simulink model "PMSM_Simulation_2025a"  (R2025a)
settings: Solver=FixedStepDiscrete  StartTime=0.0  StopTime=10  FixedStep=0.00005/200  RelTol=1e-3
values from neighbouring files (symbols this model uses):
  MC_DCurrLopKi_CFG = 0.008293758    [PMSM_MC_Data_2025a.sldd]
  MC_DCurrLopKp_CFG = 0.0870848    [PMSM_MC_Data_2025a.sldd]
  MC_MotModeDebug_CFG = 255.0    [PMSM_MC_Data_2025a.sldd]
  MC_POLE_NUM_CFG = 7.0    [PMSM_MC_Data_2025a.sldd]
  MC_QCurrLopKi_CFG = 0.008293758    [PMSM_MC_Data_2025a.sldd]
  MC_QCurrLopKp_CFG = 0.0870848    [PMSM_MC_Data_2025a.sldd]
  MC_SpdLopKi_CFG = 1.0E-5    [PMSM_MC_Data_2025a.sldd]
  MC_SpdLopKp_CFG = 0.002    [PMSM_MC_Data_2025a.sldd]
undefined symbols (not defined in the file or in its folder): Ls, magnitude, Rs
libraries: simulink x28, slpidlib x6, spsDCVoltageSourceLib x1, spsPermanentMagnetSynchronousMachineLib x1, spsUniversalBridgeLib x1, sps_lib x1
(part 1 of 3)
settings Model: DataDictionary=PMSM_MC_Data_2025a.sldd  SimulationMode=accelerator  PacingRate=1000  Creator=EDY  LastModifiedBy=xiaoy
settings RTWCC: GPUComputeCapability=3.5

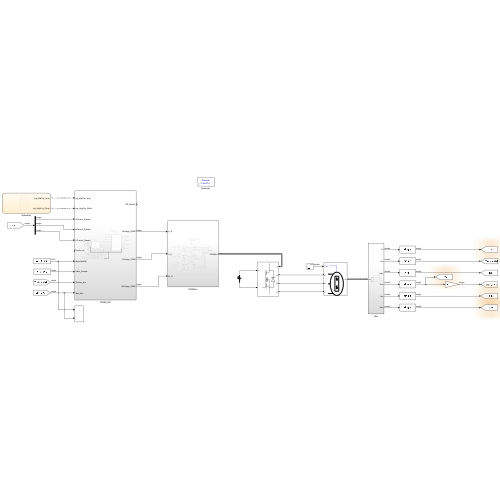
[thumbnail: Simulink's stored preview of the top-level diagram]
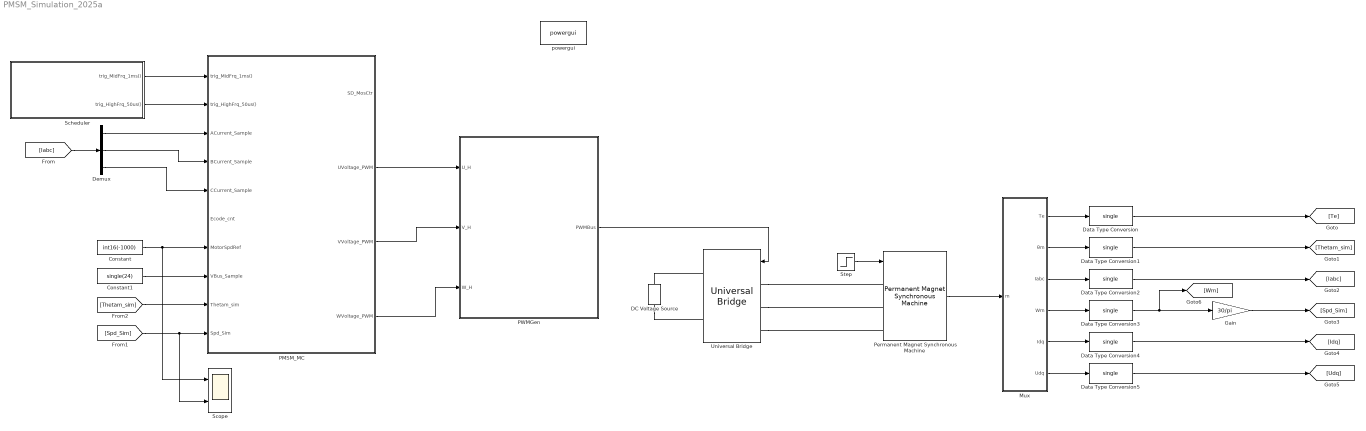
== system PMSM_Simulation_2025a ==
  Constant : Constant  Value=int16(-1000)
  Constant1 : Constant  Value=single(24)
  DC Voltage Source : spsDCVoltageSourceLib/DC Voltage Source  Amplitude=24  Measurements=None
  Data Type Conversion{,1..5} (6 alike) : DataTypeConversion  OutDataTypeStr=single  SaturateOnIntegerOverflow=off  RndMeth=Floor
  Demux : Demux  Outputs=3
  Gain : Gain  Gain=30/pi
  Mux : Subsystem
  PMSM_MC : Subsystem
  PWMGen : Subsystem
  Permanent Magnet Synchronous Machine : spsPermanentMagnetSynchronousMachineLib/Permanent Magnet Synchronous Machine  NbPhases=3  FluxDistribution=Sinusoidal  RotorType=Salient-pole  MechanicalLoad=Torque Tm  PresetModel=No  ShowDetailedParameters=on  MeasurementBus=off  Resistance=0.08  Inductance=8.5e-3  dqInductances=[0.000042,0.000042]  La=0.000395  MachineConstant=Flux linkage established by magnets (V.s)  Flux=0.00838  VoltageCst=10.6397  TorqueCst=0.08799  Flat=120  Mechanical=[0.000008 0 7 0]  PolePairs=4  InitialConditions=[0,0, 0,0]  InitialConditions5ph=[0 0 0 0 0 0]  RefAngle=Aligned with phase A axis (original Park)  IterativeDiscreteModel=Trapezoidal non iterative  TsBlock=-1  TsPowergui=0
  Scheduler : Stateflow chart  TreatAsAtomicUnit=on
  Scope : Scope  NumInputPorts=2
      settings: ActiveDisplayYMinimum=-1203.7366380691528  ActiveDisplayYMaximum=224.12290668487546
  Step : Step  Time=0  After=0  SampleTime=0
  Universal Bridge : spsUniversalBridgeLib/Universal Bridge  Arms=3  SnubberResistance=1e5  SnubberCapacitance=inf  Device=MOSFET / Diodes  Ron=1e-3  Lon=0  ForwardVoltages="[  0  0  ]"  ForwardVoltage=0  GTOparameters=[ 10e-6 , 20e-6 ]  IGBTparameters=[ 1e-6 , 2e-6 ]  Measurements=None  Measurements_2=None  converterType=Rectifier
  powergui : sps_lib/powergui  Priority=1  SimulationMode=Discrete  SampleTime=0.00005/200  frequency=60  Iterations=50  frequencyindice=0  Pbase=100e6  ErrMax=1e-4  UnitsV=kV  UnitsW=MW  buscounter=0  FunctionMessages=off  echomessages=off  EnableUseOfTLC=off  CurrentSourceSwitches=off  DisableSnubberDevices=off  DisableRonSwitches=off  DisableVfSwitches=off  DisplayEquations=off  AutomaticDiscreteSolvers=off  SolverType=Tustin/Backward Euler (TBE)  Interpol=off  ExternalGateDelay=off  methode=off  Ts=100  x0status=blocks  SPID=on  SwTol=0  HookPort=off  NonlinearTolerance=1e-4  nMaxIteration=100  ContinueOnMaxIteration=off  RestoreLinks=warning  ResistiveCurrentMeasurement=off  Frange=[0:2:500]  Ylog=off  Xlog=on  ShowGrid=off  save=off  variable=ZData  structure=0  ZoomFFT=off  StartTime=0.0  cycles=1  DisplayStyle=1  fundamental=60  FreqAxis=off  MaxFrequency=1000  frequencyindicesteady=1  RmsSteady=1  display=off
  wires:
  Step/1 -> Permanent Magnet Synchronous Machine/1
  Scheduler/1(trig_MidFrq_1ms()) -> PMSM_MC/1(trig_MidFrq_1ms())
  Scheduler/2(trig_HighFrq_50us()) -> PMSM_MC/2(trig_HighFrq_50us())
  PMSM_MC/2(UVoltage_PWM) -> PWMGen/1(U_H)
  PMSM_MC/3(VVoltage_PWM) -> PWMGen/2(V_H)
  PMSM_MC/4(WVoltage_PWM) -> PWMGen/3(W_H)
  PWMGen/1(PWMBus) -> Universal Bridge/1
  Permanent Magnet Synchronous Machine/1 -> Mux/1(m)
  Mux/1(Te) -> Data Type Conversion/1
  Mux/2(θm) -> Data Type Conversion1/1
  Mux/3(Iabc) -> Data Type Conversion2/1
  Mux/4(Wm) -> Data Type Conversion3/1
  Mux/5(Idq) -> Data Type Conversion4/1
  Mux/6(Udq) -> Data Type Conversion5/1
  Data Type Conversion/1 -> [Te]
  Data Type Conversion1/1 -> [Thetam_sim]
  Data Type Conversion2/1 -> [Iabc]
  Data Type Conversion3/1 -> Gain/1, [Wm]
  Gain/1 -> [Spd_Sim]
  Data Type Conversion4/1 -> [Idq]
  Data Type Conversion5/1 -> [Udq]
  Demux/1 -> PMSM_MC/3(ACurrent_Sample)
  Demux/2 -> PMSM_MC/4(BCurrent_Sample)
  Demux/3 -> PMSM_MC/5(CCurrent_Sample)
  [Iabc] -> Demux/1
  Constant/1 -> Scope/1, PMSM_MC/7(MotorSpdRef)
  Constant1/1 -> PMSM_MC/8(VBus_Sample)
  [Thetam_sim] -> PMSM_MC/9(Thetam_sim)
  [Spd_Sim] -> Scope/2, PMSM_MC/10(Spd_Sim)
  connections:
  Universal Bridge/LConn1 -- Permanent Magnet Synchronous Machine/LConn1
  Universal Bridge/LConn2 -- Permanent Magnet Synchronous Machine/LConn2
  Universal Bridge/LConn3 -- Permanent Magnet Synchronous Machine/LConn3
  DC Voltage Source/LConn1 -- Universal Bridge/RConn2
  DC Voltage Source/RConn1 -- Universal Bridge/RConn1

== system PMSM_Simulation_2025a/Mux ==
  m : Inport
  Bus Selector : BusSelector  OutputSignals=Stator current is_a (A),Stator current is_b (A),Stator current is_c (A),Stator voltage Vs_d (V),Stator voltage Vs_q (V),Stator current is_d (A),Stator current is_q (A)
  Bus Selector1 : BusSelector  OutputSignals=Rotor speed wm (rad/s),Rotor angle thetam (rad),Electromagnetic torque Te (N*m)
  Mux : Mux  Inputs=3
  Mux1 : Mux  Inputs=2
  Mux2 : Mux  Inputs=2
  Te : Outport
  θm : Outport  Port=2
  Iabc : Outport  Port=3
  Wm : Outport  Port=4
  Idq : Outport  Port=5
  Udq : Outport  Port=6
  wires:
  m/1 -> Bus Selector1/1, Bus Selector/1
  Bus Selector/1 -> Mux/1  "<Stator current is_a (A)>"
  Bus Selector/2 -> Mux/2  "<Stator current is_b (A)>"
  Bus Selector/3 -> Mux/3  "<Stator current is_c (A)>"
  Bus Selector/5 -> Mux1/2  "<Stator voltage Vs_q (V)>"
  Bus Selector/4 -> Mux1/1  "<Stator voltage Vs_d (V)>"
  Bus Selector/6 -> Mux2/1  "<Stator current is_d (A)>"
  Bus Selector/7 -> Mux2/2  "<Stator current is_q (A)>"
  Mux/1 -> Iabc/1
  Mux1/1 -> Udq/1
  Mux2/1 -> Idq/1
  Bus Selector1/1 -> Wm/1  "<Rotor speed wm (rad/s)>"
  Bus Selector1/2 -> θm/1  "<Rotor angle thetam (rad)>"
  Bus Selector1/3 -> Te/1  "<Electromagnetic torque Te (N*m)>"

== system PMSM_Simulation_2025a/PMSM_MC ==
  trig_MidFrq_1ms() : Inport
  trig_HighFrq_50us() : Inport  Port=2
  ACurrent_Sample : Inport  Port=3
  BCurrent_Sample : Inport  Port=4
  CCurrent_Sample : Inport  Port=5
  Ecode_cnt : Inport  Port=6
  MotorSpdRef : Inport  Port=7
  VBus_Sample : Inport  Port=8
  Thetam_sim : Inport  Port=9
  Spd_Sim : Inport  Port=10
  Add : Sum  Inputs=+-
  Atan2 : Trigonometry  Operator=atan2
  Bus Selector : BusSelector  OutputSignals=Thetae_Est
  Constant3 : Constant  Value=single(2*pi)
  Cos : Trigonometry  Operator=cos
  Gain : Gain  Gain=7
  MC_HighFrqTask : Subsystem  TreatAsAtomicUnit=on
  MC_LowFrqTask : Subsystem  TreatAsAtomicUnit=on
  Mod : Math  Operator=mod
  Scope : Scope  NumInputPorts=2
      settings: ActiveDisplayYMinimum=-0.78539818525314309  ActiveDisplayYMaximum=7.06858366727829  DataLoggingVariableName=ScopeData12
  Sin : Trigonometry
  theta_erro : Scope
      settings: ActiveDisplayYMinimum=-2.4846426397562027  ActiveDisplayYMaximum=7.2573886066675186  DataLoggingVariableName=ScopeData9
  SD_MosCtr : Outport
  UVoltage_PWM : Outport  Port=2
  VVoltage_PWM : Outport  Port=3
  WVoltage_PWM : Outport  Port=4
  wires:
  trig_HighFrq_50us()/1 -> MC_HighFrqTask/Trigger
  Ecode_cnt/1 -> MC_LowFrqTask/2(Ecode_cnt), MC_HighFrqTask/9(Ecode_cnt)
  MotorSpdRef/1 -> MC_LowFrqTask/1(MotorSpdRef), MC_HighFrqTask/11(MotorSpdRef)
  ACurrent_Sample/1 -> MC_HighFrqTask/1(ACurrent_Sample)
  BCurrent_Sample/1 -> MC_HighFrqTask/2(BCurrent_Sample)
  CCurrent_Sample/1 -> MC_HighFrqTask/3(CCurrent_Sample)
  VBus_Sample/1 -> MC_HighFrqTask/4(VBus_Sample)
  MC_LowFrqTask/1(QAxiCurrent_Ref) -> MC_HighFrqTask/5(QAxiCurrent_Ref)
  MC_LowFrqTask/2(MotCalThetae) -> MC_HighFrqTask/6(MotCalThetae)
  MC_LowFrqTask/3(MotOffset) -> MC_HighFrqTask/7(MotOffset)
  MC_LowFrqTask/4(MotCtrMode) -> MC_HighFrqTask/8(MotCtrMode)
  MC_HighFrqTask/1(SD_MosCtr) -> SD_MosCtr/1
  MC_HighFrqTask/2(UVoltage_PWM) -> UVoltage_PWM/1
  MC_HighFrqTask/3(VVoltage_PWM) -> VVoltage_PWM/1
  MC_HighFrqTask/4(WVoltage_PWM) -> WVoltage_PWM/1
  Spd_Sim/1 -> MC_LowFrqTask/3(Spd_Sim)
  trig_MidFrq_1ms()/1 -> MC_LowFrqTask/Trigger
  Thetam_sim/1 -> Gain/1, MC_HighFrqTask/10(Thetam_sim)
  MC_HighFrqTask/5(OLStartCompletedFlag) -> MC_LowFrqTask/4(OLStartCompletedFlag)
  MC_HighFrqTask/6(FOCBusInfo) -> Bus Selector/1, MC_LowFrqTask/5(FOCBusInfo)
  Bus Selector/1 -> Add/2, Scope/2  "<Thetae_Est>"
  Constant3/1 -> Mod/2
  Gain/1 -> Mod/1
  Mod/1 -> Scope/1, Add/1
  Add/1 -> Sin/1, Cos/1
  Sin/1 -> Atan2/1
  Cos/1 -> Atan2/2
  Atan2/1 -> theta_erro/1

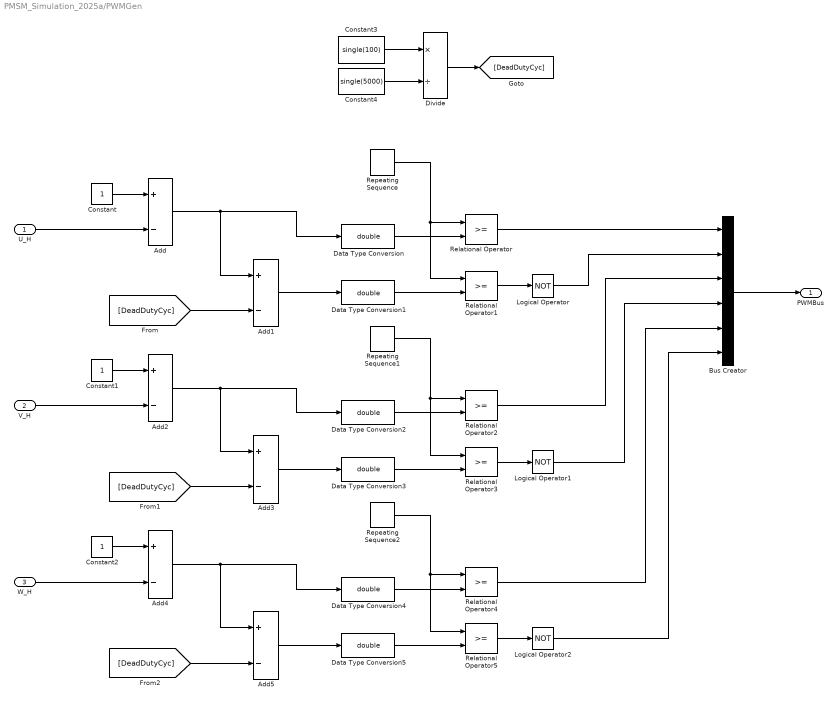
== system PMSM_Simulation_2025a/PWMGen ==
  U_H : Inport
  V_H : Inport  Port=2
  W_H : Inport  Port=3
  Add{,1..5} (6 alike) : Sum  Inputs=+-
  Bus Creator : BusCreator  Inputs=6
  Constant : Constant
  Constant1 : Constant
  Constant2 : Constant
  Constant3 : Constant  Value=single(100)
  Constant4 : Constant  Value=single(5000)
  Data Type Conversion{,1..5} (6 alike) : DataTypeConversion  OutDataTypeStr=double  SaturateOnIntegerOverflow=off  RndMeth=Floor
  Divide : Product  Inputs=*/
  Logical Operator : Logic  Operator=NOT  AllPortsSameDT=off  OutDataTypeStr=boolean
  Logical Operator1 : Logic  Operator=NOT  AllPortsSameDT=off  OutDataTypeStr=boolean
  Logical Operator2 : Logic  Operator=NOT  AllPortsSameDT=off  OutDataTypeStr=boolean
  Relational Operator{,1..5} (6 alike) : RelationalOperator  OutDataTypeStr=boolean  RndMeth=Simplest  InputSameDT=off
  Repeating Sequence : simulink/Sources/Repeating Sequence  rep_seq_t=[0 0.00005/2 0.00005]  rep_seq_y=[0 1 0]
  Repeating Sequence1 : simulink/Sources/Repeating Sequence  rep_seq_t=[0 0.00005/2 0.00005]  rep_seq_y=[0 1 0]
  Repeating Sequence2 : simulink/Sources/Repeating Sequence  rep_seq_t=[0 0.00005/2 0.00005]  rep_seq_y=[0 1 0]
  PWMBus : Outport
  wires:
  Constant/1 -> Add/1
  U_H/1 -> Add/2
  Add/1 -> Add1/1, Data Type Conversion/1
  Add1/1 -> Data Type Conversion1/1
  Data Type Conversion/1 -> Relational Operator/2
  Repeating Sequence/1 -> Relational Operator1/1, Relational Operator/1
  Data Type Conversion1/1 -> Relational Operator1/2
  Relational Operator1/1 -> Logical Operator/1
  Data Type Conversion2/1 -> Relational Operator2/2
  Repeating Sequence1/1 -> Relational Operator3/1, Relational Operator2/1
  Add2/1 -> Add3/1, Data Type Conversion2/1
  Data Type Conversion3/1 -> Relational Operator3/2
  V_H/1 -> Add2/2
  Add3/1 -> Data Type Conversion3/1
  Relational Operator3/1 -> Logical Operator1/1
  Constant1/1 -> Add2/1
  Constant2/1 -> Add4/1
  Relational Operator5/1 -> Logical Operator2/1
  Add4/1 -> Add5/1, Data Type Conversion4/1
  Repeating Sequence2/1 -> Relational Operator5/1, Relational Operator4/1
  Data Type Conversion4/1 -> Relational Operator4/2
  Data Type Conversion5/1 -> Relational Operator5/2
  Add5/1 -> Data Type Conversion5/1
  W_H/1 -> Add4/2
  Relational Operator/1 -> Bus Creator/1
  Logical Operator/1 -> Bus Creator/2
  Relational Operator2/1 -> Bus Creator/3
  Logical Operator1/1 -> Bus Creator/4
  Relational Operator4/1 -> Bus Creator/5
  Logical Operator2/1 -> Bus Creator/6
  Bus Creator/1 -> PWMBus/1
  Constant3/1 -> Divide/1
  Constant4/1 -> Divide/2
  Divide/1 -> [DeadDutyCyc]
  [DeadDutyCyc] -> Add1/2
  [DeadDutyCyc] -> Add3/2
  [DeadDutyCyc] -> Add5/2

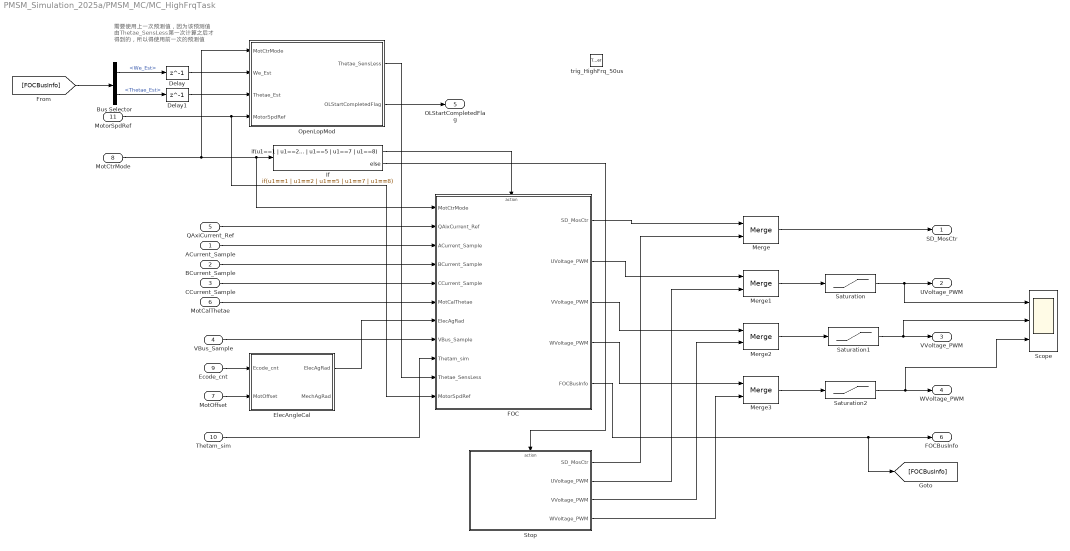
== system PMSM_Simulation_2025a/PMSM_MC/MC_HighFrqTask ==
  note: 需要使用上一次预测值，因为该预测值
      | 由Thetae_SensLess第一次计算之后才
      | 得到的，所以得使用前一次的预测值
  ACurrent_Sample : Inport
  BCurrent_Sample : Inport  Port=2
  CCurrent_Sample : Inport  Port=3
  VBus_Sample : Inport  Port=4
  QAxiCurrent_Ref : Inport  Port=5
  MotCalThetae : Inport  Port=6
  MotOffset : Inport  Port=7
  MotCtrMode : Inport  Port=8
  Ecode_cnt : Inport  Port=9
  Thetam_sim : Inport  Port=10
  MotorSpdRef : Inport  Port=11
  trig_HighFrq_50us : TriggerPort  TriggerType=function-call  VariantControl=(inherit)
  Bus Selector : BusSelector  OutputSignals=We_Est,Thetae_Est
  Delay : Delay  DelayLength=1
  Delay1 : Delay  DelayLength=1
  ElecAngleCal : Subsystem
  FOC : Subsystem
  If : If  IfExpression=u1==1 | u1==2 | u1==5 | u1==7 | u1==8
  Merge{,1..3} (4 alike) : Merge
  OpenLopMod : Subsystem
  Saturation : Saturate  UpperLimit=0.95  LowerLimit=0
      settings: AttributesFormatString=|
      | Upper = %<UpperLimit>
      | Lower = %<LowerLimit>
  Saturation1 : Saturate  UpperLimit=0.95  LowerLimit=0
      settings: AttributesFormatString=|
      | Upper = %<UpperLimit>
      | Lower = %<LowerLimit>
  Saturation2 : Saturate  UpperLimit=0.95  LowerLimit=0
      settings: AttributesFormatString=|
      | Upper = %<UpperLimit>
      | Lower = %<LowerLimit>
  Scope : Scope  NumInputPorts=3
      settings: ActiveDisplayYMinimum=0.2183  ActiveDisplayYMaximum=0.69061
  Stop : Subsystem  TreatAsAtomicUnit=on
  SD_MosCtr : Outport
  UVoltage_PWM : Outport  Port=2
  VVoltage_PWM : Outport  Port=3
  WVoltage_PWM : Outport  Port=4
  OLStartCompletedFlag : Outport  Port=5
  FOCBusInfo : Outport  Port=6
  wires:
  MotCtrMode/1 -> If/1, FOC/1(MotCtrMode), OpenLopMod/1(MotCtrMode)
  If/1 -> FOC/Action
  If/2 -> Stop/Action
  FOC/1(SD_MosCtr) -> Merge/1
  FOC/2(UVoltage_PWM) -> Merge1/1
  FOC/3(VVoltage_PWM) -> Merge2/1
  FOC/4(WVoltage_PWM) -> Merge3/1
  Merge/1 -> SD_MosCtr/1
  Stop/1(SD_MosCtr) -> Merge/2
  Stop/2(UVoltage_PWM) -> Merge1/2
  Stop/3(VVoltage_PWM) -> Merge2/2
  Stop/4(WVoltage_PWM) -> Merge3/2
  Merge1/1 -> Saturation/1
  Merge3/1 -> Saturation2/1
  Merge2/1 -> Saturation1/1
  Saturation/1 -> UVoltage_PWM/1, Scope/1
  Saturation1/1 -> Scope/2, VVoltage_PWM/1
  Saturation2/1 -> Scope/3, WVoltage_PWM/1
  MotOffset/1 -> ElecAngleCal/2(MotOffset)
  Ecode_cnt/1 -> ElecAngleCal/1(Ecode_cnt)
  ACurrent_Sample/1 -> FOC/3(ACurrent_Sample)
  BCurrent_Sample/1 -> FOC/4(BCurrent_Sample)
  CCurrent_Sample/1 -> FOC/5(CCurrent_Sample)
  QAxiCurrent_Ref/1 -> FOC/2(QAixCurrent_Ref)
  MotCalThetae/1 -> FOC/6(MotCalThetae)
  VBus_Sample/1 -> FOC/8(VBus_Sample)
  ElecAngleCal/1(ElecAgRad) -> FOC/7(ElecAgRad)
  Thetam_sim/1 -> FOC/9(Thetam_sim)
  OpenLopMod/2(OLStartCompletedFlag) -> OLStartCompletedFlag/1
  MotorSpdRef/1 -> FOC/11(MotorSpdRef), OpenLopMod/4(MotorSpdRef)
  OpenLopMod/1(Thetae_SensLess) -> FOC/10(Thetae_SensLess)
  FOC/5(FOCBusInfo) -> [FOCBusInfo], FOCBusInfo/1
  [FOCBusInfo] -> Bus Selector/1
  Bus Selector/1 -> Delay/1  "<We_Est>"
  Bus Selector/2 -> Delay1/1  "<Thetae_Est>"
  Delay/1 -> OpenLopMod/2(We_Est)
  Delay1/1 -> OpenLopMod/3(Thetae_Est)

== system PMSM_Simulation_2025a/PMSM_MC/MC_LowFrqTask ==
  note: 此处的We_Est不需要使用delay模块
      | 是因为在高频任务产生，等该低频任务
      | 调用时已经存在值了，所以就不会报错
  MotorSpdRef : Inport
  Ecode_cnt : Inport  Port=2
  Spd_Sim : Inport  Port=3
  OLStartCompletedFlag : Inport  Port=4
  FOCBusInfo : Inport  Port=5
  trig_MidFrq_1ms : TriggerPort  TriggerType=function-call  VariantControl=(inherit)
  Bus Selector : BusSelector  OutputSignals=We_Est
  MotModeCtr : Subsystem
  MotSpdCal : Subsystem
  SpdLoop : Subsystem
  QAxiCurrent_Ref : Outport
  MotCalThetae : Outport  Port=2
  MotOffset : Outport  Port=3
  MotCtrMode : Outport  Port=4
  wires:
  SpdLoop/1(QAxiCurrent_Ref) -> QAxiCurrent_Ref/1
  MotorSpdRef/1 -> SpdLoop/2(MotorSpdRef), MotModeCtr/2(MotorSpdRef)
  Ecode_cnt/1 -> MotSpdCal/1(Ecode_cnt), MotModeCtr/1(Ecode_cnt)
  MotModeCtr/3(MotCtrMode) -> MotCtrMode/1, SpdLoop/1(MotCtrMode)
  MotModeCtr/2(MotCalThetae) -> MotCalThetae/1
  MotModeCtr/1(MotOffset) -> MotOffset/1
  OLStartCompletedFlag/1 -> MotModeCtr/3(OLStartCompletedFlag)
  FOCBusInfo/1 -> Bus Selector/1
  Bus Selector/1 -> MotSpdCal/2(We_Est)  "<We_Est>"
  Spd_Sim/1 -> MotSpdCal/3(Spd_Sim)
  MotSpdCal/1(MotorActSpd) -> SpdLoop/3(MotorActSpd)

== system PMSM_Simulation_2025a/PMSM_MC/MC_HighFrqTask/ElecAngleCal ==
  Ecode_cnt : Inport
  MotOffset : Inport  Port=2
  Add : Sum  Inputs=+-
  AngleCal : Subsystem
  Demux : Demux  Outputs=2
  ElecAgRad : Outport
  MechAgRad : Outport  Port=2
  wires:
  Ecode_cnt/1 -> Add/1
  MotOffset/1 -> Add/2
  Add/1 -> AngleCal/1(Ecode_CntCorrect)
  AngleCal/1(Theta) -> Demux/1
  Demux/1 -> MechAgRad/1
  Demux/2 -> ElecAgRad/1

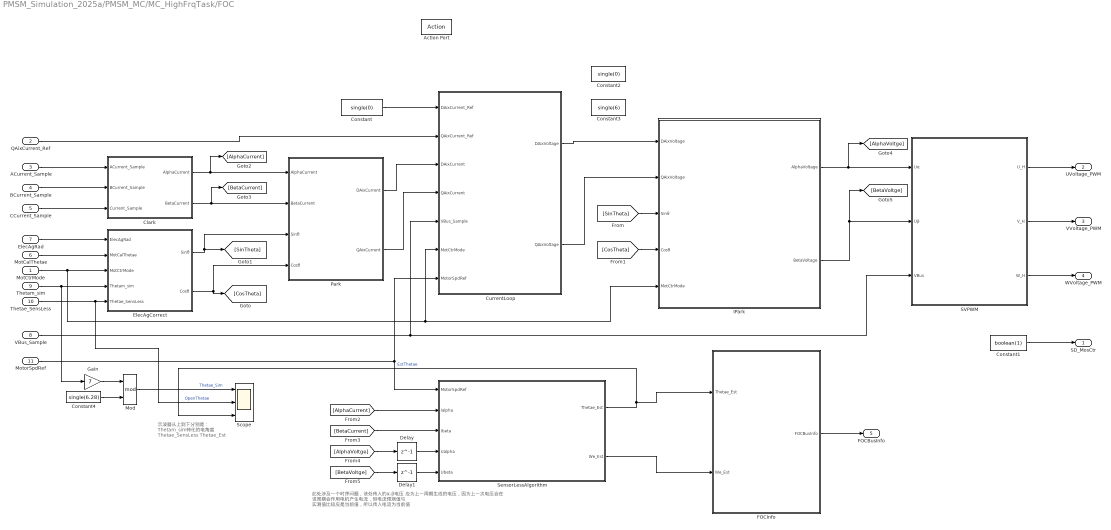
== system PMSM_Simulation_2025a/PMSM_MC/MC_HighFrqTask/FOC ==
  note: 示波器从上到下分别是：
      | Thetam_sim转化的电角度
      | Thetae_SensLess
      | Thetae_Est
  note: 此处涉及一个时序问题，该处传入的α-β电压
      | 应为上一周期生成的电压，因为上一次电压会在
      | 该周期会作用电机产生电流，但电流预测值与
      | 实测值比较应是当前值，所以传入电流为当前值
  MotCtrMode : Inport
  QAixCurrent_Ref : Inport  Port=2
  ACurrent_Sample : Inport  Port=3
  BCurrent_Sample : Inport  Port=4
  CCurrent_Sample : Inport  Port=5
  MotCalThetae : Inport  Port=6
  ElecAgRad : Inport  Port=7
  VBus_Sample : Inport  Port=8
  Thetam_sim : Inport  Port=9
  Thetae_SensLess : Inport  Port=10
  MotorSpdRef : Inport  Port=11
  Action Port : ActionPort  ActionPortLabel=if(u1==1 | u1==2 | u1==5 | u1==7 | u1==8)
  Clark : Subsystem
  Constant : Constant  Value=single(0)
  Constant1 : Constant  Value=boolean(1)
  Constant2 : Constant  Value=single(0)
  Constant3 : Constant  Value=single(6)
  Constant4 : Constant  Value=single(6.28)
  CurrentLoop : Subsystem
  Delay : Delay  DelayLength=1
  Delay1 : Delay  DelayLength=1
  ElecAgCorrect : Subsystem
  FOCInfo : Subsystem
  Gain : Gain  Gain=7
  IPark : Subsystem
  Mod : Math  Operator=mod
  Park : Subsystem
  SVPWM : Subsystem
  Scope : Scope  NumInputPorts=3
      settings: ActiveDisplayYMinimum=-0.784927427768707  ActiveDisplayYMaximum=7.0643468499183655  DataLoggingVariableName=ScopeData7
  SensorLessAlgorithm : Subsystem
  SD_MosCtr : Outport
  UVoltage_PWM : Outport  Port=2
  VVoltage_PWM : Outport  Port=3
  WVoltage_PWM : Outport  Port=4
  FOCBusInfo : Outport  Port=5
  wires:
  Clark/2(BetaCurrent) -> [BetaCurrent], Park/2(BetaCurrent)
  Clark/1(AlphaCurrent) -> [AlphaCurrent], Park/1(AlphaCurrent)
  Park/1(DAixCurrent) -> CurrentLoop/3(DAixCurrent)
  QAixCurrent_Ref/1 -> CurrentLoop/2(QAixCurrent_Ref)
  Constant/1 -> CurrentLoop/1(DAixCurrent_Ref)
  Park/2(QAixCurrent) -> CurrentLoop/4(QAixCurrent)
  ACurrent_Sample/1 -> Clark/1(ACurrent_Sample)
  BCurrent_Sample/1 -> Clark/2(BCurrent_Sample)
  CCurrent_Sample/1 -> Clark/3(Current_Sample)
  ElecAgRad/1 -> ElecAgCorrect/1(ElecAgRad)
  MotCalThetae/1 -> ElecAgCorrect/2(MotCalThetae)
  MotCtrMode/1 -> CurrentLoop/6(MotCtrMode), IPark/5(MotCtrMode), ElecAgCorrect/3(MotCtrMode)
  ElecAgCorrect/1(Sinθ) -> Park/3(Sinθ), [SinTheta]
  ElecAgCorrect/2(Cosθ) -> [CosTheta], Park/4(Cosθ)
  [SinTheta] -> IPark/3(Sinθ)
  [CosTheta] -> IPark/4(Cosθ)
  VBus_Sample/1 -> CurrentLoop/5(VBus_Sample), SVPWM/3(VBus)
  IPark/1(AlphaVoltage) -> [AlphaVoltge], SVPWM/1(Uα)
  IPark/2(BetaVoltage) -> [BetaVoltge], SVPWM/2(Uβ)
  SVPWM/1(U_H) -> UVoltage_PWM/1
  SVPWM/2(V_H) -> VVoltage_PWM/1
  SVPWM/3(W_H) -> WVoltage_PWM/1
  Constant1/1 -> SD_MosCtr/1
  Thetam_sim/1 -> ElecAgCorrect/4(Thetam_sim), Gain/1
  CurrentLoop/1(DAixVoltage) -> IPark/1(DAixVoltage)
  CurrentLoop/2(QAixVoltage) -> IPark/2(QAixVoltage)
  Thetae_SensLess/1 -> Scope/2, ElecAgCorrect/5(Thetae_SensLess)  "OpenThetae"
  MotorSpdRef/1 -> SensorLessAlgorithm/1(MotorSpdRef), CurrentLoop/7(MotorSpdRef)
  [BetaVoltge] -> Delay1/1
  [AlphaVoltge] -> Delay/1
  [BetaCurrent] -> SensorLessAlgorithm/3(Ibeta)
  [AlphaCurrent] -> SensorLessAlgorithm/2(Ialpha)
  Delay/1 -> SensorLessAlgorithm/4(Ualpha)
  Delay1/1 -> SensorLessAlgorithm/5(Ubeta)
  SensorLessAlgorithm/1(Thetae_Est) -> Scope/3, FOCInfo/1(Thetae_Est)  "EstThetae"
  SensorLessAlgorithm/2(We_Est) -> FOCInfo/2(We_Est)
  FOCInfo/1(FOCBusInfo) -> FOCBusInfo/1
  Gain/1 -> Mod/1
  Constant4/1 -> Mod/2
  Mod/1 -> Scope/1  "Thetae_Sim"

== system PMSM_Simulation_2025a/PMSM_MC/MC_HighFrqTask/OpenLopMod ==
  note: 加权切换时间
  note: 每个周期只允许增加机械1rpm，也需要
      | 换算为电气的rad/s
  note: OLSpdRef_rpm为开环的机械目标转速
      | 需要将机械rpm转化为电速度rad/s
  note: Thetae_Est为观测器电角度，需要
      | 将输入角度归一化到[0 2pi]的角度输出
  note: 注意输入的We_Est是电角速度，
      | 状态机里面的是机械角速度
  MotCtrMode : Inport
  We_Est : Inport  Port=2
  Thetae_Est : Inport  Port=3
  MotorSpdRef : Inport  Port=4
  AngleNormalization : Subsystem
  Divide : Product  Inputs=*/
  Gain : Gain  Gain=2*pi*7/60
  Gain1 : Gain  Gain=2*pi*7/60
  Gain2 : Gain  Gain=2*pi/60
  Gain3 : Gain  Gain=1000/50
  OLSpdRampMaxStep_rpm : Constant  Value=single(1)
  OLSpdRef_rpm : Constant  Value=single(300)
  OLSpdStableThd_rpm : Constant  Value=single(200)
  OLSpdStableTime_ms : Constant  Value=single(100)
  OLWeightedTransmTime_ms : Constant  Value=single(0.1)
  OpenLopThetaeCal : Stateflow chart  TreatAsAtomicUnit=on
  Pn : Constant  Value=single(7)
  Ts : Constant  Value=single(0.00005)
  Thetae_SensLess : Outport
  OLStartCompletedFlag : Outport  Port=2
  wires:
  MotCtrMode/1 -> OpenLopThetaeCal/1(MotCtrMode)
  Divide/1 -> OpenLopThetaeCal/2(Wm_Est)
  We_Est/1 -> Divide/1
  Pn/1 -> Divide/2
  AngleNormalization/1(ThetaNorm) -> OpenLopThetaeCal/3(Thetae_Est)
  Thetae_Est/1 -> AngleNormalization/1(Theta)
  MotorSpdRef/1 -> OpenLopThetaeCal/4(MotorSpdRef)
  Gain/1 -> OpenLopThetaeCal/5(OLWeRef)
  OLSpdRampMaxStep_rpm/1 -> Gain1/1
  Gain1/1 -> OpenLopThetaeCal/6(OLWeRampMaxStep)
  OLSpdStableThd_rpm/1 -> Gain2/1
  Gain2/1 -> OpenLopThetaeCal/7(OLSpdStableThd)
  Gain3/1 -> OpenLopThetaeCal/8(OLSpdStableCnt)
  OLSpdStableTime_ms/1 -> Gain3/1
  Ts/1 -> OpenLopThetaeCal/9(Ts)
  OLWeightedTransmTime_ms/1 -> OpenLopThetaeCal/10(OLWeightedTransmTime)
  OpenLopThetaeCal/2(OLStartCompletedFlag) -> OLStartCompletedFlag/1
  OpenLopThetaeCal/1(Thetae_SensLess) -> Thetae_SensLess/1
  OLSpdRef_rpm/1 -> Gain/1

== system PMSM_Simulation_2025a/PMSM_MC/MC_HighFrqTask/Stop ==
  Action Port : ActionPort  ActionPortLabel=else
  Constant : Constant  Value=single(0)
  Constant1 : Constant  Value=boolean(0)
  SD_MosCtr : Outport
  UVoltage_PWM : Outport  Port=2
  VVoltage_PWM : Outport  Port=3
  WVoltage_PWM : Outport  Port=4
  wires:
  Constant/1 -> WVoltage_PWM/1, VVoltage_PWM/1, UVoltage_PWM/1
  Constant1/1 -> SD_MosCtr/1

== system PMSM_Simulation_2025a/PMSM_MC/MC_LowFrqTask/MotModeCtr ==
  Ecode_cnt : Inport
  MotorSpdRef : Inport  Port=2
  OLStartCompletedFlag : Inport  Port=3
  Compare To Constant : simulink/Logic and Bit Operations/Compare To Constant  relop=~=  const=255  OutDataTypeStr=boolean
  Constant : Constant  Value=MC_MotModeDebug_CFG
  Constant1 : Constant  Value=boolean(1)
  Constant2 : Constant  Value=boolean(0)
  ModeMgr : Stateflow chart  TreatAsAtomicUnit=on
  Switch : Switch  Criteria=u2 ~= 0  SaturateOnIntegerOverflow=off  InputSameDT=off
  MotOffset : Outport
  MotCalThetae : Outport  Port=2
  MotCtrMode : Outport  Port=3
  wires:
  ModeMgr/2(MotOffset) -> MotOffset/1
  ModeMgr/3(MotCalThetae) -> MotCalThetae/1
  Ecode_cnt/1 -> ModeMgr/1(Ecode_cnt)
  MotorSpdRef/1 -> ModeMgr/2(MotorSpdRef)
  ModeMgr/1(MotCtrMode) -> Switch/3
  Switch/1 -> MotCtrMode/1
  Constant/1 -> Switch/1, Compare To Constant/1
  Compare To Constant/1 -> Switch/2
  Constant1/1 -> ModeMgr/3(SensorLessEn)
  Constant2/1 -> ModeMgr/4(OpenLoopEn)
  OLStartCompletedFlag/1 -> ModeMgr/5(OLStartCompletedFlag)

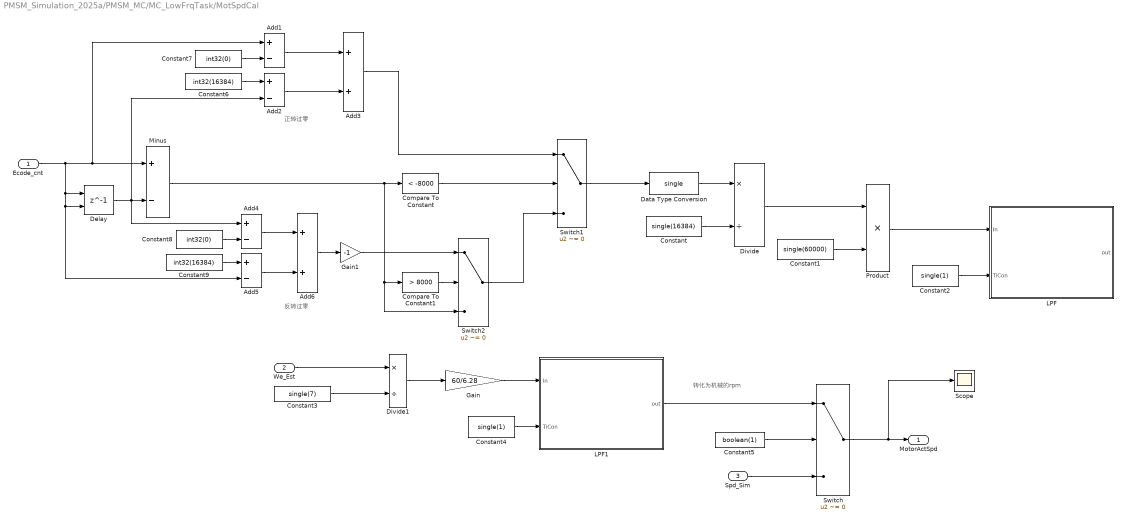
== system PMSM_Simulation_2025a/PMSM_MC/MC_LowFrqTask/MotSpdCal ==
  note: 正转过零
  note: 转化为机械的rpm
  note: 反转过零
  Ecode_cnt : Inport
  We_Est : Inport  Port=2
  Spd_Sim : Inport  Port=3
  Add{1..2,4..5} (4 alike) : Sum  Inputs=+-
  Add3 : Sum
  Add6 : Sum
  Compare To Constant : simulink/Logic and Bit Operations/Compare To Constant  relop=<  const=-8000  OutDataTypeStr=boolean
  Compare To Constant1 : simulink/Logic and Bit Operations/Compare To Constant  relop=>  const=8000  OutDataTypeStr=boolean
  Constant : Constant  Value=single(16384)
  Constant1 : Constant  Value=single(60000)
  Constant2 : Constant  Value=single(1)
  Constant3 : Constant  Value=single(7)
  Constant4 : Constant  Value=single(1)
  Constant5 : Constant  Value=boolean(1)
  Constant6 : Constant  Value=int32(16384)
  Constant7 : Constant  Value=int32(0)
  Constant8 : Constant  Value=int32(0)
  Constant9 : Constant  Value=int32(16384)
  Data Type Conversion : DataTypeConversion  OutDataTypeStr=single  SaturateOnIntegerOverflow=off  RndMeth=Floor
  Delay : Delay  DelayLength=1  InitialConditionSource=Input port
      settings: InputPortMap=u0,p4
  Divide : Product  Inputs=*/
  Divide1 : Product  Inputs=*/
  Gain : Gain  Gain=60/6.28
  Gain1 : Gain  Gain=-1
  LPF : Subsystem
  LPF1 : Subsystem
  Minus : Sum  Inputs=+-
  Product : Product
  Scope : Scope
      settings: ActiveDisplayYMinimum=-5893.0649108886719  ActiveDisplayYMaximum=17858.338592529297  DataLoggingVariableName=ScopeData14
  Switch : Switch  Criteria=u2 ~= 0  SaturateOnIntegerOverflow=off  InputSameDT=off
  Switch1 : Switch  Criteria=u2 ~= 0  SaturateOnIntegerOverflow=off  InputSameDT=off
  Switch2 : Switch  Criteria=u2 ~= 0  SaturateOnIntegerOverflow=off  InputSameDT=off
  MotorActSpd : Outport
  wires:
  Ecode_cnt/1 -> Add5/2, Delay/2, Delay/1, Add1/1, Minus/1
  Delay/1 -> Add4/1, Add2/2, Minus/2
  Data Type Conversion/1 -> Divide/1
  Constant/1 -> Divide/2
  Divide/1 -> Product/1
  Constant1/1 -> Product/2
  Product/1 -> LPF/1(In)
  Constant2/1 -> LPF/2(TiCon)
  We_Est/1 -> Divide1/1
  Constant3/1 -> Divide1/2
  Divide1/1 -> Gain/1
  Gain/1 -> LPF1/1(In)
  Constant4/1 -> LPF1/2(TiCon)
  LPF1/1(out) -> Switch/1
  Constant5/1 -> Switch/2
  Spd_Sim/1 -> Switch/3
  Switch/1 -> Scope/1, MotorActSpd/1
  Add1/1 -> Add3/1
  Add3/1 -> Switch1/1
  Gain1/1 -> Switch2/1
  Add5/1 -> Add6/2
  Add6/1 -> Gain1/1
  Minus/1 -> Compare To Constant/1, Compare To Constant1/1, Switch2/3
  Switch2/1 -> Switch1/3
  Add4/1 -> Add6/1
  Add2/1 -> Add3/2
  Compare To Constant/1 -> Switch1/2
  Constant7/1 -> Add1/2
  Constant6/1 -> Add2/1
  Compare To Constant1/1 -> Switch2/2
  Constant8/1 -> Add4/2
  Constant9/1 -> Add5/1
  Switch1/1 -> Data Type Conversion/1

== system PMSM_Simulation_2025a/PMSM_MC/MC_LowFrqTask/SpdLoop ==
  MotCtrMode : Inport
  MotorSpdRef : Inport  Port=2
  MotorActSpd : Inport  Port=3
  Compare To Constant : simulink/Logic and Bit Operations/Compare To Constant  relop===  const=5  OutDataTypeStr=boolean
  Constant : Constant  Value=single(0)  OutDataTypeStr=single
  Constant1 : Constant  Value=single(3)
  Constant2 : Constant  Value=MC_SpdLopKp_CFG
  Constant3 : Constant  Value=MC_SpdLopKi_CFG
  Constant4 : Constant  Value=int16(2000)
  Data Type Conversion : DataTypeConversion  OutDataTypeStr=single  SaturateOnIntegerOverflow=off  RndMeth=Floor
  Discrete PID Controller : slpidlib/PID Controller  Controller=PI  Form=Parallel  TimeDomain=Discrete-time  UseExternalTs=off  SampleTime=-1  IntegratorMethod=Forward Euler  FilterMethod=Forward Euler  ControllerParametersSource=external  P=1  I=1  UseKiTs=on  D=0  UseExternalDerivativeSource=off  N=100  UseFilter=on  TunerSelectOption=Transfer Function Based (PID Tuner App)  InitialConditionSource=external  InitialConditionForIntegrator=0  InitialConditionForFilter=0  DifferentiatorICPrevScaledInput=0  ExternalReset=rising  TrackingMode=off  Kt=1  LimitOutput=off  SatLimitsSource=external  UpperSaturationLimit=inf  LowerSaturationLimit=-inf  LinearizeAsGain=off  AntiWindupMode=none  Kb=1  LimitIntegrator=on  UpperIntegratorSaturationLimit=3  LowerIntegratorSaturationLimit=-3  POutMin=[]  POutMax=[]  IOutMin=[]  IOutMax=[]  DOutMin=[]  DOutMax=[]  NOutMin=[]  NOutMax=[]  SumOutMin=[]  SumOutMax=[]  SaturationOutMin=[]  SaturationOutMax=[]  PParamMin=[]  PParamMax=[]  IParamMin=[]  IParamMax=[]  DParamMin=[]  DParamMax=[]  NParamMin=[]  NParamMax=[]  KbParamMin=[]  KbParamMax=[]  KtParamMin=[]  KtParamMax=[]  KbOutMin=[]  KbOutMax=[]  KtOutMin=[]  KtOutMax=[]  IntegratorOutMin=[]  IntegratorOutMax=[]  FilterOutMin=[]  FilterOutMax=[]  SumI1OutMin=[]  SumI1OutMax=[]  SumI2OutMin=[]  SumI2OutMax=[]  SumI3OutMin=[]  SumI3OutMax=[]  SumI4OutMin=[]  SumI4OutMax=[]  SumDOutMin=[]  SumDOutMax=[]  DifferentiatorOutMin=[]  DifferentiatorOutMax=[]  FilterDiffOutCoefMin=[]  FilterDiffOutCoefMax=[]  ReciprocalOutMin=[]  ReciprocalOutMax=[]  SumDenOutMin=[]  SumDenOutMax=[]  SumNumOutMin=[]  SumNumOutMax=[]  DivideOutMin=[]  DivideOutMax=[]  UdiffTsProdOutMin=[]  UdiffTsProdOutMax=[]  NTsProdOutMin=[]  NTsProdOutMax=[]  UintegralTsProdOutMin=[]  UintegralTsProdOutMax=[]  UngainTsProdOutMin=[]  UngainTsProdOutMax=[]  ClampingZeroOutDataTypeStr=Inherit: Inherit via back propagation  ClampingZeroOutMin=[]  ClampingZeroOutMax=[]  FilterDenConstantOutDataTypeStr=Inherit: Inherit via back propagation  FilterDenConstantOutMin=[]  FilterDenConstantOutMax=[]  PCopyOutDataTypeStr=Inherit: Inherit via back propagation  PCopyOutMin=[]  PCopyOutMax=[]  NCopyOutDataTypeStr=Inherit: Inherit via back propagation  NCopyOutMin=[]  NCopyOutMax=[]  IntegratorContinuousStateAttributes=''  IntegratorStateMustResolveToSignalObject=off  IntegratorRTWStateStorageClass=Auto  FilterContinuousStateAttributes=''  FilterStateMustResolveToSignalObject=off  FilterRTWStateStorageClass=Auto  ParallelPVariant=ExternalParameters  IdealPVariant=Disabled  IVariant=ExternalParameters  DVariant=Disabled  IntegratorVariant=Discrete  SatVariant=Disabled  AWVariant=Passthrough  PCopyVariant=Disabled  TRVariant=Disabled  FdbkBlocksVariant=Forward  IdealPFdbkVariant=Disabled  SatFdbkVariant=Disabled  DerivativeFilterVariant=Disabled  NVariant=Disabled  NCopyVariant=Disabled_SignalSpec  FilterICVariant=Disabled  IntegratorICVariant=ExternalICs  ExternalResetVariant=ExternalReset  TRSumVariant=Passthrough  SumFdbkVariant=Disabled  SumVariant=Sum_PI  TsampFilterVariant=InternalTs  TsampNgainVariant=Passthrough  TsampIntegralVariant=Disabled_SignalSpec  ExternalSaturationOutDataTypeStr=Inherit: Same as second input  DerivativeSourceVariant=Disabled  PreIntVariant=InternalPreInt
      settings: LibrarySourceBlock=simulink/Discrete/Discrete PID Controller
  Gain : Gain  Gain=-1
  Gain1 : Gain  Gain=-1
  Minus : Sum  Inputs=+-
  Saturation Dynamic : simulink/Discontinuities/Saturation Dynamic  OutMin=[]  OutMax=[]  OutDataTypeStr=Inherit: Same as second input  OutDataType=fixdt(1, 16)  OutScaling=2^-10  DoSatur=off
  Saturation Dynamic1 : simulink/Discontinuities/Saturation Dynamic  OutMin=[]  OutMax=[]  OutDataTypeStr=Inherit: Same as second input  OutDataType=fixdt(1, 16)  OutScaling=2^-10  DoSatur=off
  QAxiCurrent_Ref : Outport
  wires:
  Data Type Conversion/1 -> Minus/1
  Constant/1 -> Discrete PID Controller/5
  Discrete PID Controller/1 -> Saturation Dynamic/2
  Saturation Dynamic/1 -> QAxiCurrent_Ref/1
  Constant1/1 -> Saturation Dynamic/1, Gain/1
  Gain/1 -> Saturation Dynamic/3
  Minus/1 -> Discrete PID Controller/1
  Constant2/1 -> Discrete PID Controller/2
  Constant3/1 -> Discrete PID Controller/3
  MotorSpdRef/1 -> Saturation Dynamic1/2
  Saturation Dynamic1/1 -> Data Type Conversion/1
  Constant4/1 -> Gain1/1, Saturation Dynamic1/1
  Gain1/1 -> Saturation Dynamic1/3
  MotorActSpd/1 -> Minus/2
  Compare To Constant/1 -> Discrete PID Controller/4
  MotCtrMode/1 -> Compare To Constant/1

== system PMSM_Simulation_2025a/PMSM_MC/MC_HighFrqTask/ElecAngleCal/AngleCal ==
  Ecode_CntCorrect : Inport
  If : If  IfExpression=u1 == 1  ElseIfExpressions=u1 == -1
  If Action Subsystem : Subsystem  TreatAsAtomicUnit=on
  If Action Subsystem1 : Subsystem  TreatAsAtomicUnit=on
  If Action Subsystem2 : Subsystem  TreatAsAtomicUnit=on
  Merge : Merge  Inputs=3
  Sign : Signum
  Theta : Outport
  wires:
  Ecode_CntCorrect/1 -> If Action Subsystem1/1(Ecode_PhyVal), If Action Subsystem/1(Ecode_PhyVal), Sign/1
  Sign/1 -> If/1
  If/1 -> If Action Subsystem/Action
  If/2 -> If Action Subsystem1/Action
  If/3 -> If Action Subsystem2/Action
  If Action Subsystem1/1(Out1) -> Merge/2
  If Action Subsystem/1(Out1) -> Merge/1
  Merge/1 -> Theta/1
  If Action Subsystem2/1(Out1) -> Merge/3

== system PMSM_Simulation_2025a/PMSM_MC/MC_HighFrqTask/FOC/Clark ==
  ACurrent_Sample : Inport
  BCurrent_Sample : Inport  Port=2
  Current_Sample : Inport  Port=3
  Gain : Gain  Gain=0.57735
  Gain1 : Gain  Gain=0.57735
  Minus : Sum  Inputs=+-
  AlphaCurrent : Outport
  BetaCurrent : Outport  Port=2
  wires:
  ACurrent_Sample/1 -> AlphaCurrent/1
  Minus/1 -> BetaCurrent/1
  Gain1/1 -> Minus/2
  Gain/1 -> Minus/1
  BCurrent_Sample/1 -> Gain/1
  Current_Sample/1 -> Gain1/1

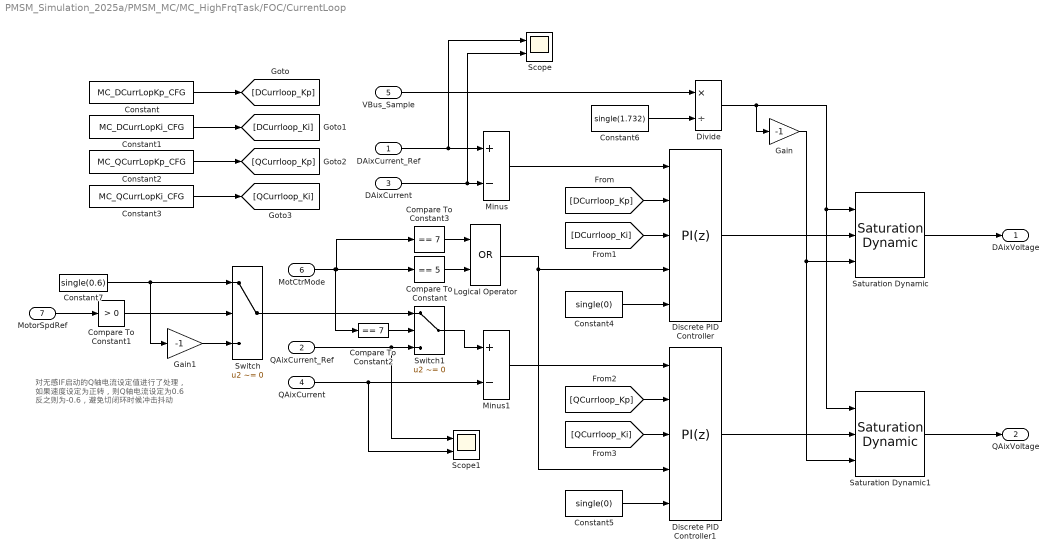
== system PMSM_Simulation_2025a/PMSM_MC/MC_HighFrqTask/FOC/CurrentLoop ==
  note: 对无感IF启动的Q轴电流设定值进行了处理，
      | 如果速度设定为正转，则Q轴电流设定为0.6
      | 反之则为-0.6，避免切闭环时候冲击抖动
  DAixCurrent_Ref : Inport
  QAixCurrent_Ref : Inport  Port=2
  DAixCurrent : Inport  Port=3
  QAixCurrent : Inport  Port=4
  VBus_Sample : Inport  Port=5
  MotCtrMode : Inport  Port=6
  MotorSpdRef : Inport  Port=7
  Compare To Constant : simulink/Logic and Bit Operations/Compare To Constant  relop===  const=5  OutDataTypeStr=boolean
  Compare To Constant1 : simulink/Logic and Bit Operations/Compare To Constant  relop=>  const=0  OutDataTypeStr=boolean
  Compare To Constant2 : simulink/Logic and Bit Operations/Compare To Constant  relop===  const=7  OutDataTypeStr=boolean
  Compare To Constant3 : simulink/Logic and Bit Operations/Compare To Constant  relop===  const=7  OutDataTypeStr=boolean
  Constant : Constant  Value=MC_DCurrLopKp_CFG
  Constant1 : Constant  Value=MC_DCurrLopKi_CFG
  Constant2 : Constant  Value=MC_QCurrLopKp_CFG
  Constant3 : Constant  Value=MC_QCurrLopKi_CFG
  Constant4 : Constant  Value=single(0)
  Constant5 : Constant  Value=single(0)
  Constant6 : Constant  Value=single(1.732)
  Constant7 : Constant  Value=single(0.6)
  Discrete PID Controller : slpidlib/PID Controller  Controller=PI  Form=Parallel  TimeDomain=Discrete-time  UseExternalTs=off  SampleTime=-1  IntegratorMethod=Forward Euler  FilterMethod=Forward Euler  ControllerParametersSource=external  P=1  I=1  UseKiTs=on  D=0  UseExternalDerivativeSource=off  N=100  UseFilter=on  TunerSelectOption=Transfer Function Based (PID Tuner App)  InitialConditionSource=external  InitialConditionForIntegrator=0  InitialConditionForFilter=0  DifferentiatorICPrevScaledInput=0  ExternalReset=rising  TrackingMode=off  Kt=1  LimitOutput=off  SatLimitsSource=internal  UpperSaturationLimit=inf  LowerSaturationLimit=-inf  LinearizeAsGain=off  AntiWindupMode=none  Kb=1  LimitIntegrator=on  UpperIntegratorSaturationLimit=13  LowerIntegratorSaturationLimit=-13  POutMin=[]  POutMax=[]  IOutMin=[]  IOutMax=[]  DOutMin=[]  DOutMax=[]  NOutMin=[]  NOutMax=[]  SumOutMin=[]  SumOutMax=[]  SaturationOutMin=[]  SaturationOutMax=[]  PParamMin=[]  PParamMax=[]  IParamMin=[]  IParamMax=[]  DParamMin=[]  DParamMax=[]  NParamMin=[]  NParamMax=[]  KbParamMin=[]  KbParamMax=[]  KtParamMin=[]  KtParamMax=[]  KbOutMin=[]  KbOutMax=[]  KtOutMin=[]  KtOutMax=[]  IntegratorOutMin=[]  IntegratorOutMax=[]  FilterOutMin=[]  FilterOutMax=[]  SumI1OutMin=[]  SumI1OutMax=[]  SumI2OutMin=[]  SumI2OutMax=[]  SumI3OutMin=[]  SumI3OutMax=[]  SumI4OutMin=[]  SumI4OutMax=[]  SumDOutMin=[]  SumDOutMax=[]  DifferentiatorOutMin=[]  DifferentiatorOutMax=[]  FilterDiffOutCoefMin=[]  FilterDiffOutCoefMax=[]  ReciprocalOutMin=[]  ReciprocalOutMax=[]  SumDenOutMin=[]  SumDenOutMax=[]  SumNumOutMin=[]  SumNumOutMax=[]  DivideOutMin=[]  DivideOutMax=[]  UdiffTsProdOutMin=[]  UdiffTsProdOutMax=[]  NTsProdOutMin=[]  NTsProdOutMax=[]  UintegralTsProdOutMin=[]  UintegralTsProdOutMax=[]  UngainTsProdOutMin=[]  UngainTsProdOutMax=[]  ClampingZeroOutDataTypeStr=Inherit: Inherit via back propagation  ClampingZeroOutMin=[]  ClampingZeroOutMax=[]  FilterDenConstantOutDataTypeStr=Inherit: Inherit via back propagation  FilterDenConstantOutMin=[]  FilterDenConstantOutMax=[]  PCopyOutDataTypeStr=Inherit: Inherit via back propagation  PCopyOutMin=[]  PCopyOutMax=[]  NCopyOutDataTypeStr=Inherit: Inherit via back propagation  NCopyOutMin=[]  NCopyOutMax=[]  IntegratorContinuousStateAttributes=''  IntegratorStateMustResolveToSignalObject=off  IntegratorRTWStateStorageClass=Auto  FilterContinuousStateAttributes=''  FilterStateMustResolveToSignalObject=off  FilterRTWStateStorageClass=Auto  ParallelPVariant=ExternalParameters  IdealPVariant=Disabled  IVariant=ExternalParameters  DVariant=Disabled  IntegratorVariant=Discrete  SatVariant=Disabled  AWVariant=Passthrough  PCopyVariant=Disabled  TRVariant=Disabled  FdbkBlocksVariant=Forward  IdealPFdbkVariant=Disabled  SatFdbkVariant=Disabled  DerivativeFilterVariant=Disabled  NVariant=Disabled  NCopyVariant=Disabled_SignalSpec  FilterICVariant=Disabled  IntegratorICVariant=ExternalICs  ExternalResetVariant=ExternalReset  TRSumVariant=Passthrough  SumFdbkVariant=Disabled  SumVariant=Sum_PI  TsampFilterVariant=InternalTs  TsampNgainVariant=Passthrough  TsampIntegralVariant=Disabled_SignalSpec  ExternalSaturationOutDataTypeStr=Inherit: Same as second input  DerivativeSourceVariant=Disabled  PreIntVariant=InternalPreInt
      settings: LibrarySourceBlock=simulink/Discrete/Discrete PID Controller
  Discrete PID Controller1 : slpidlib/PID Controller  Controller=PI  Form=Parallel  TimeDomain=Discrete-time  UseExternalTs=off  SampleTime=-1  IntegratorMethod=Forward Euler  FilterMethod=Forward Euler  ControllerParametersSource=external  P=1  I=1  UseKiTs=on  D=0  UseExternalDerivativeSource=off  N=100  UseFilter=on  TunerSelectOption=Transfer Function Based (PID Tuner App)  InitialConditionSource=external  InitialConditionForIntegrator=0  InitialConditionForFilter=0  DifferentiatorICPrevScaledInput=0  ExternalReset=rising  TrackingMode=off  Kt=1  LimitOutput=off  SatLimitsSource=internal  UpperSaturationLimit=inf  LowerSaturationLimit=-inf  LinearizeAsGain=off  AntiWindupMode=none  Kb=1  LimitIntegrator=on  UpperIntegratorSaturationLimit=13  LowerIntegratorSaturationLimit=-13  POutMin=[]  POutMax=[]  IOutMin=[]  IOutMax=[]  DOutMin=[]  DOutMax=[]  NOutMin=[]  NOutMax=[]  SumOutMin=[]  SumOutMax=[]  SaturationOutMin=[]  SaturationOutMax=[]  PParamMin=[]  PParamMax=[]  IParamMin=[]  IParamMax=[]  DParamMin=[]  DParamMax=[]  NParamMin=[]  NParamMax=[]  KbParamMin=[]  KbParamMax=[]  KtParamMin=[]  KtParamMax=[]  KbOutMin=[]  KbOutMax=[]  KtOutMin=[]  KtOutMax=[]  IntegratorOutMin=[]  IntegratorOutMax=[]  FilterOutMin=[]  FilterOutMax=[]  SumI1OutMin=[]  SumI1OutMax=[]  SumI2OutMin=[]  SumI2OutMax=[]  SumI3OutMin=[]  SumI3OutMax=[]  SumI4OutMin=[]  SumI4OutMax=[]  SumDOutMin=[]  SumDOutMax=[]  DifferentiatorOutMin=[]  DifferentiatorOutMax=[]  FilterDiffOutCoefMin=[]  FilterDiffOutCoefMax=[]  ReciprocalOutMin=[]  ReciprocalOutMax=[]  SumDenOutMin=[]  SumDenOutMax=[]  SumNumOutMin=[]  SumNumOutMax=[]  DivideOutMin=[]  DivideOutMax=[]  UdiffTsProdOutMin=[]  UdiffTsProdOutMax=[]  NTsProdOutMin=[]  NTsProdOutMax=[]  UintegralTsProdOutMin=[]  UintegralTsProdOutMax=[]  UngainTsProdOutMin=[]  UngainTsProdOutMax=[]  ClampingZeroOutDataTypeStr=Inherit: Inherit via back propagation  ClampingZeroOutMin=[]  ClampingZeroOutMax=[]  FilterDenConstantOutDataTypeStr=Inherit: Inherit via back propagation  FilterDenConstantOutMin=[]  FilterDenConstantOutMax=[]  PCopyOutDataTypeStr=Inherit: Inherit via back propagation  PCopyOutMin=[]  PCopyOutMax=[]  NCopyOutDataTypeStr=Inherit: Inherit via back propagation  NCopyOutMin=[]  NCopyOutMax=[]  IntegratorContinuousStateAttributes=''  IntegratorStateMustResolveToSignalObject=off  IntegratorRTWStateStorageClass=Auto  FilterContinuousStateAttributes=''  FilterStateMustResolveToSignalObject=off  FilterRTWStateStorageClass=Auto  ParallelPVariant=ExternalParameters  IdealPVariant=Disabled  IVariant=ExternalParameters  DVariant=Disabled  IntegratorVariant=Discrete  SatVariant=Disabled  AWVariant=Passthrough  PCopyVariant=Disabled  TRVariant=Disabled  FdbkBlocksVariant=Forward  IdealPFdbkVariant=Disabled  SatFdbkVariant=Disabled  DerivativeFilterVariant=Disabled  NVariant=Disabled  NCopyVariant=Disabled_SignalSpec  FilterICVariant=Disabled  IntegratorICVariant=ExternalICs  ExternalResetVariant=ExternalReset  TRSumVariant=Passthrough  SumFdbkVariant=Disabled  SumVariant=Sum_PI  TsampFilterVariant=InternalTs  TsampNgainVariant=Passthrough  TsampIntegralVariant=Disabled_SignalSpec  ExternalSaturationOutDataTypeStr=Inherit: Same as second input  DerivativeSourceVariant=Disabled  PreIntVariant=InternalPreInt
      settings: LibrarySourceBlock=simulink/Discrete/Discrete PID Controller
  Divide : Product  Inputs=*/
  Gain : Gain  Gain=-1
  Gain1 : Gain  Gain=-1
  Logical Operator : Logic  Operator=OR  AllPortsSameDT=off  OutDataTypeStr=boolean
  Minus : Sum  Inputs=+-
  Minus1 : Sum  Inputs=+-
  Saturation Dynamic : simulink/Discontinuities/Saturation Dynamic  OutMin=[]  OutMax=[]  OutDataTypeStr=Inherit: Same as second input  OutDataType=fixdt(1, 16)  OutScaling=2^-10  DoSatur=off
  Saturation Dynamic1 : simulink/Discontinuities/Saturation Dynamic  OutMin=[]  OutMax=[]  OutDataTypeStr=Inherit: Same as second input  OutDataType=fixdt(1, 16)  OutScaling=2^-10  DoSatur=off
  Scope : Scope  NumInputPorts=2
      settings: ActiveDisplayYMinimum=-1  ActiveDisplayYMaximum=1  DataLoggingVariableName=ScopeData16
  Scope1 : Scope  NumInputPorts=2
      settings: ActiveDisplayYMinimum=-1  ActiveDisplayYMaximum=1  DataLoggingVariableName=ScopeData17
  Switch : Switch  Criteria=u2 ~= 0  SaturateOnIntegerOverflow=off  InputSameDT=off
  Switch1 : Switch  Criteria=u2 ~= 0  SaturateOnIntegerOverflow=off  InputSameDT=off
  DAixVoltage : Outport
  QAixVoltage : Outport  Port=2
  wires:
  Minus/1 -> Discrete PID Controller/1
  DAixCurrent_Ref/1 -> Minus/1, Scope/1
  DAixCurrent/1 -> Scope/2, Minus/2
  QAixCurrent/1 -> Minus1/2, Scope1/2
  QAixCurrent_Ref/1 -> Scope1/1, Switch1/3
  Minus1/1 -> Discrete PID Controller1/1
  Constant/1 -> [DCurrloop_Kp]
  Constant1/1 -> [DCurrloop_Ki]
  Constant2/1 -> [QCurrloop_Kp]
  Constant3/1 -> [QCurrloop_Ki]
  [DCurrloop_Kp] -> Discrete PID Controller/2
  [DCurrloop_Ki] -> Discrete PID Controller/3
  Constant4/1 -> Discrete PID Controller/5
  [QCurrloop_Kp] -> Discrete PID Controller1/2
  [QCurrloop_Ki] -> Discrete PID Controller1/3
  Constant5/1 -> Discrete PID Controller1/5
  Constant6/1 -> Divide/2
  VBus_Sample/1 -> Divide/1
  Divide/1 -> Gain/1, Saturation Dynamic1/1, Saturation Dynamic/1
  Discrete PID Controller/1 -> Saturation Dynamic/2
  Discrete PID Controller1/1 -> Saturation Dynamic1/2
  Saturation Dynamic/1 -> DAixVoltage/1
  Saturation Dynamic1/1 -> QAixVoltage/1
  Gain/1 -> Saturation Dynamic1/3, Saturation Dynamic/3
  MotCtrMode/1 -> Compare To Constant2/1, Compare To Constant3/1, Compare To Constant/1
  MotorSpdRef/1 -> Compare To Constant1/1
  Compare To Constant1/1 -> Switch/2
  Gain1/1 -> Switch/3
  Constant7/1 -> Switch/1, Gain1/1
  Switch/1 -> Switch1/1
  Compare To Constant2/1 -> Switch1/2
  Switch1/1 -> Minus1/1
  Compare To Constant3/1 -> Logical Operator/1
  Compare To Constant/1 -> Logical Operator/2
  Logical Operator/1 -> Discrete PID Controller/4, Discrete PID Controller1/4

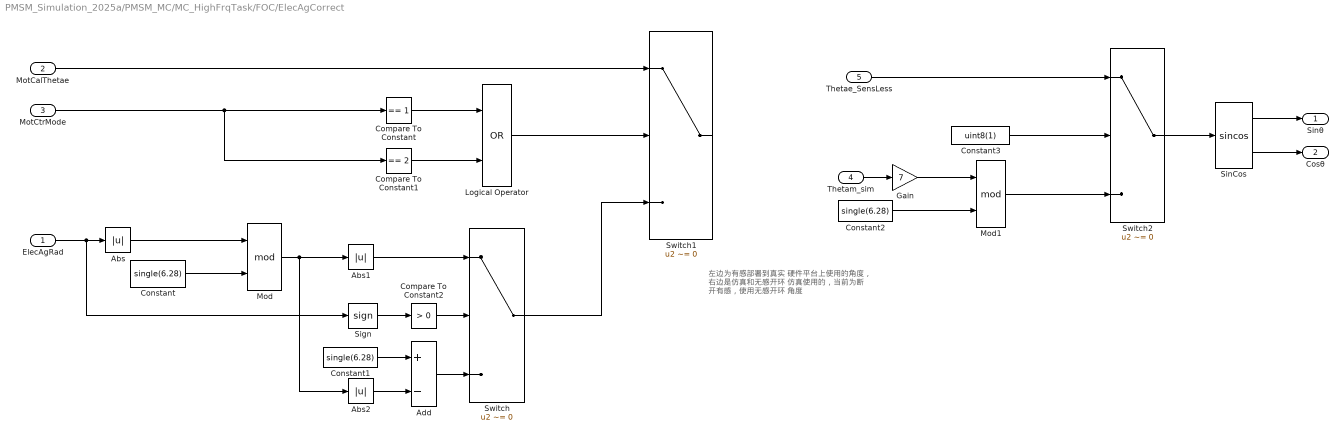
== system PMSM_Simulation_2025a/PMSM_MC/MC_HighFrqTask/FOC/ElecAgCorrect ==
  note: 左边为有感部署到真实
      | 硬件平台上使用的角度，
      | 右边是仿真和无感开环
      | 仿真使用的，当前为断
      | 开有感，使用无感开环
      | 角度
  ElecAgRad : Inport
  MotCalThetae : Inport  Port=2
  MotCtrMode : Inport  Port=3
  Thetam_sim : Inport  Port=4
  Thetae_SensLess : Inport  Port=5
  Abs : Abs  SaturateOnIntegerOverflow=off
  Abs1 : Abs  SaturateOnIntegerOverflow=off
  Abs2 : Abs  SaturateOnIntegerOverflow=off
  Add : Sum  Inputs=+-
  Compare To Constant : simulink/Logic and Bit Operations/Compare To Constant  relop===  const=1  OutDataTypeStr=boolean
  Compare To Constant1 : simulink/Logic and Bit Operations/Compare To Constant  relop===  const=2  OutDataTypeStr=boolean
  Compare To Constant2 : simulink/Logic and Bit Operations/Compare To Constant  relop=>  const=0  OutDataTypeStr=boolean
  Constant : Constant  Value=single(6.28)
  Constant1 : Constant  Value=single(6.28)
  Constant2 : Constant  Value=single(6.28)
  Constant3 : Constant  Value=uint8(1)
  Gain : Gain  Gain=7
  Logical Operator : Logic  Operator=OR  AllPortsSameDT=off  OutDataTypeStr=boolean
  Mod : Math  Operator=mod
  Mod1 : Math  Operator=mod
  Sign : Signum
  SinCos : Trigonometry  Operator=sincos
  Switch : Switch  Criteria=u2 ~= 0  SaturateOnIntegerOverflow=off  InputSameDT=off
  Switch1 : Switch  Criteria=u2 ~= 0  SaturateOnIntegerOverflow=off  InputSameDT=off
  Switch2 : Switch  Criteria=u2 ~= 0  SaturateOnIntegerOverflow=off  InputSameDT=off
  Sinθ : Outport
  Cosθ : Outport  Port=2
  wires:
  ElecAgRad/1 -> Abs/1, Sign/1
  Constant/1 -> Mod/2
  Abs/1 -> Mod/1
  Mod/1 -> Abs2/1, Abs1/1
  MotCtrMode/1 -> Compare To Constant1/1, Compare To Constant/1
  Compare To Constant/1 -> Logical Operator/1
  Compare To Constant1/1 -> Logical Operator/2
  Sign/1 -> Compare To Constant2/1
  Compare To Constant2/1 -> Switch/2
  Abs1/1 -> Switch/1
  Logical Operator/1 -> Switch1/2
  MotCalThetae/1 -> Switch1/1
  SinCos/1 -> Sinθ/1
  SinCos/2 -> Cosθ/1
  Switch/1 -> Switch1/3
  Add/1 -> Switch/3
  Constant1/1 -> Add/1
  Abs2/1 -> Add/2
  Thetam_sim/1 -> Gain/1
  Thetae_SensLess/1 -> Switch2/1
  Mod1/1 -> Switch2/3
  Gain/1 -> Mod1/1
  Constant2/1 -> Mod1/2
  Constant3/1 -> Switch2/2
  Switch2/1 -> SinCos/1

== system PMSM_Simulation_2025a/PMSM_MC/MC_HighFrqTask/FOC/FOCInfo ==
  Thetae_Est : Inport
  We_Est : Inport  Port=2
  Bus Creator : BusCreator  Inputs=2
  FOCBusInfo : Outport
  wires:
  Thetae_Est/1 -> Bus Creator/1  "Thetae_Est"
  We_Est/1 -> Bus Creator/2  "We_Est"
  Bus Creator/1 -> FOCBusInfo/1  "FOCBusInfo"

== system PMSM_Simulation_2025a/PMSM_MC/MC_HighFrqTask/FOC/IPark ==
  note: 一共有8种电机运行模式，其中1，2为电机零位标定，
      | 3为标定失败，4表示Stop模式，5代表有感启动正常运行，
      | 6为无感启动失败模式，7为IF启动，8为VF启动模式
  DAixVoltage : Inport
  QAixVoltage : Inport  Port=2
  Sinθ : Inport  Port=3
  Cosθ : Inport  Port=4
  MotCtrMode : Inport  Port=5
  Add : Sum
  Constant : Constant  Value=single(0)
  Constant1 : Constant  Value=single(0)
  Constant2 : Constant  Value=single(1)
  Constant3 : Constant  Value=single(1)
  Minus : Sum  Inputs=+-
  Multiport Switch : MultiPortSwitch  Inputs=8  DiagnosticForDefault=None  SaturateOnIntegerOverflow=off  InputSameDT=off
  Multiport Switch1 : MultiPortSwitch  Inputs=8  DiagnosticForDefault=None  SaturateOnIntegerOverflow=off  InputSameDT=off
  Product{1..4} (4 alike) : Product
  AlphaVoltage : Outport
  BetaVoltage : Outport  Port=2
  wires:
  Multiport Switch/1 -> Product4/1, Product3/1
  Cosθ/1 -> Product4/2, Product1/1
  Sinθ/1 -> Product3/2, Product2/2
  Multiport Switch1/1 -> Product1/2, Product2/1
  Product4/1 -> Minus/1
  Product2/1 -> Minus/2
  Minus/1 -> AlphaVoltage/1
  Product1/1 -> Add/1
  MotCtrMode/1 -> Multiport Switch1/1, Multiport Switch/1
  QAixVoltage/1 -> Multiport Switch1/8, Multiport Switch1/6
  DAixVoltage/1 -> Multiport Switch/8, Multiport Switch/6
  Product3/1 -> Add/2
  Add/1 -> BetaVoltage/1
  Constant1/1 -> Multiport Switch/9, Multiport Switch/7, Multiport Switch/5, Multiport Switch/4
  Constant/1 -> Multiport Switch1/4, Multiport Switch1/3, Multiport Switch1/2, Multiport Switch1/5, Multiport Switch1/7
  Constant3/1 -> Multiport Switch/3, Multiport Switch/2
  Constant2/1 -> Multiport Switch1/9

== system PMSM_Simulation_2025a/PMSM_MC/MC_HighFrqTask/FOC/Park ==
  AlphaCurrent : Inport
  BetaCurrent : Inport  Port=2
  Sinθ : Inport  Port=3
  Cosθ : Inport  Port=4
  Add : Sum
  Add1 : Sum  Inputs=+-
  Product{,1..3} (4 alike) : Product
  DAixCurrent : Outport
  QAixCurrent : Outport  Port=2
  wires:
  Cosθ/1 -> Product2/1, Product/2
  BetaCurrent/1 -> Product1/1, Product2/2
  Sinθ/1 -> Product3/2, Product1/2
  AlphaCurrent/1 -> Product3/1, Product/1
  Product/1 -> Add/1
  Product1/1 -> Add/2
  Add/1 -> DAixCurrent/1
  Product2/1 -> Add1/1
  Product3/1 -> Add1/2
  Add1/1 -> QAixCurrent/1

== system PMSM_Simulation_2025a/PMSM_MC/MC_HighFrqTask/FOC/SVPWM ==
  Uα : Inport
  Uβ : Inport  Port=2
  VBus : Inport  Port=3
  SevenSegSVPWM : Subsystem
  U_H : Outport
  V_H : Outport  Port=2
  W_H : Outport  Port=3
  wires:
  Uα/1 -> SevenSegSVPWM/1(Uα)
  Uβ/1 -> SevenSegSVPWM/2(Uβ)
  VBus/1 -> SevenSegSVPWM/3(VBus)
  SevenSegSVPWM/1(UVoltage_PWM) -> U_H/1
  SevenSegSVPWM/2(VVoltage_PWM) -> V_H/1
  SevenSegSVPWM/3(WVoltage_PWM) -> W_H/1
